simulink model "IEEE_BUS_68_Baseline"  (R2025a)
settings: Solver=ode23tb  StartTime=0.0  StopTime=150  FixedStep=Ts  MaxStep=0.0001  RelTol=1e-3
PreLoadFcn:
  | PSSMODEL=1;
  | LPSS=0;
  | WAPSS=0;
  | WAPSS2=0;
  | Ts=50e-5;
InitFcn:
  | PSSMODEL=1;
  | LPSS=0;
  | WAPSS=0;
  | WAPSS2=0;
  | Ts=50e-5;
  | 
  | % Required data to 68 Bus benchmark
  | % clear
  | % clc
  | % Definition for the columns
  | % system base =100 MVA
  | 
  | %% Line data Format (line)
  | % All values are given on the same system base MVA
  | % 1: From bus
  | % 2: To bus
  | % 3: Resistance (pu)
  | % 4: Reactance  (pu)
  | % 5: Charge     (pu)
  | % 6: Transformer Tap Amplitute
  | % 7: base MVA
  | % 8: Nomonal Voltage (KV)
  | 
  | %1   2    3        4       5       6        7      8
  | line=[...
  | 1	54	0	     0.0181	  0	      1.025     100    13.8
  | 2	58	0	     0.025	  0	      1.070     100    13.8
  | 3	62	0	     0.02	  0	      1.070     100    13.8
  | 4	19	0.0007	 0.0142	  0	      1.070     100    13.8
  | 5	20	0.0009	 0.018	  0	      1.009     100    13.8
  | 6	22	0	     0.0143	  0	      1.025     100    13.8
  | 7	23	0.0005	 0.0272	  0	      0         100    13.8
  | 8	25	0.0006	 0.0232	  0	      1.025     100    13.8
  | 9	29	0.0008	 0.0156   0	      1.025     100    13.8
  | 10	31	0	     0.026	  0	      1.04      100    13.8
  | 11	32	0	     0.013	  0	      1.04      100    13.8
  | 12	36	0	     0.0075	  0	      1.04      100    13.8
  | 13	17	0	     0.0033	  0	      1.04      100    13.8
  | 14	41	0	     0.0015	  0	      1         100    13.8
  | 15	42	0	     0.0015	  0	      1         100    13.8
  | 16	18	0	     0.003	  0	      1         100    13.8
  | 17	36	0.0005	 0.0045	  0.32	  0         100    138
  | 17	43	0.0005	 0.0276	  0	      0         100    138
  | 18	42	0.004	 0.06	  2.25    0         100    138
  | 18	49	0.0076	 0.1141	  1.16    0	        100    138
  | 18	50	0.0012	 0.0288	  2.06	  0         100    138
  | 20	19	0.0007	 0.0138	  0       1.06	    100    138
  | 19	68	0.0016	 0.0195	  0.304	  0         100    138
  | 21	22	0.0008	 0.014	  0.2565  0	        100    138
  | 21	68	0.0008	 0.0135	  0.2548  0	        100    138
  | 22	23	0.0006	 0.0096	  0.1846  0	        100    138
  | 23	24	0.0022	 0.035	  0.361	  0         100    138
  | 24	68	0.0003	 0.0059	  0.068	  0         100    138
  | 25	26	0.0032	 0.0323	  0.531	  0         100    138
  | 25	54	0.007	 0.0086	  0.146	  0         100    138
  | 26	27	0.0014	 0.0147	  0.2396  0	        100    138
  | 26	28	0.0043	 0.0474	  0.7802  0	        100    138
  | 26	29	0.0057	 0.0625	  1.029	  0         100    138
  | 27	37	0.0013	 0.0173	  0.3216  0	        100    138
  | 27	53	0.032	 0.32	  0.41	  0         100    138
  | ... (+206 lines)
undefined symbols (not defined in the file or in its folder): D1, Delta
libraries: spsRMSLib x73, spsThreePhaseVIMeasurementLib x69, spsLoadFlowBusLib x69, spsThreePhasePISectionLineLib x64, spsThreePhaseParallelRLCLoadLib x35, spsGenericPowerSystemStabilizerLib x32, spsThreePhaseSeriesRLCLoadLib x21, spsThreePhaseTransformerTwoWindingsLib x21, spsSynchronousMachinepuStandardLib x19, spsExcitationSystemLib x16, spsMultiBandPowerSystemStabilizerLib x16, spsSteamTurbineandGovernorLib x16
(part 7 of 7)

== system IEEE_BUS_68_Baseline/area-5/G15/M15: Turbine & Regulators  ==
  note: M15
  m15 : Inport
  Pref15 : Inport  Port=2
  Vref15 : Inport  Port=3
  PSS15 : Inport  Port=4
  Bus Selector : BusSelector  OutputSignals="Mechanical.Rotor speed  wm  (pu),Mechanical.Rotor angle deviation  d_theta (rad),Mechanical.Electrical power  Pe (pu),Mechanical.Rotor speed deviation  dw (pu),Mechanical.Rotor mechanical angle  theta (deg),dq0 components.Stator voltage  vd (pu),dq0 components.Stator voltage  vq (pu),Output reactive power  Qeo (pu)"
  "Delta Pa PSS 15 " : spsGenericPowerSystemStabilizerLib/Generic Power System Stabilizer  Tsensor=15e-3  K=2.5*1.25  Twashout=1  Tleadlag1=[60e-3 1]  Tleadlag2=[0 0]  VSlimits=[-0.15 0.15]  Vinit=0  Plot_On=off  MagdB_On=on  FreqRange=logspace(-2,2,500)
      settings: LibrarySourceBlock=|
      | sps_lib/Electrical Machines/Synchronous Machine Control/Generic
      | Power System Stabilizer
  Delta w PSS (Kundur) 15 : spsGenericPowerSystemStabilizerLib/Generic Power System Stabilizer  Tsensor=15e-3  K=30  Twashout=10  Tleadlag1=[50e-3 20e-3]  Tleadlag2=[3 5.4]  VSlimits=[-0.15 0.15]  Vinit=0  Plot_On=off  MagdB_On=on  FreqRange=logspace(-2,2,500)
      settings: LibrarySourceBlock=|
      | sps_lib/Electrical Machines/Synchronous Machine Control/Generic
      | Power System Stabilizer
  EXCITATION15 : spsExcitationSystemLib/Excitation System  tr=AVR_Data(16,1)  reg=[ AVR_Data(16,2:3) ]  exc=[ 1, 0 ]  tgr=[ AVR_Data(16,4:5)]  damp=[ 0, 0 ]  sat=[ 0, 0 ]  lim="[ AVR_Data(16,7:8)  0 ]"  v0=[1 1.0005]
      settings: LibrarySourceBlock=sps_lib/Electrical Machines/Synchronous Machine Control/Excitation System
  MB-PSS15 : spsMultiBandPowerSystemStabilizerLib/Multi-Band Power System Stabilizer  OperationMode=Simplified settings  Kg=MB(1)  GL=[MB(2) MB(3)]  GI=[MB(4) MB(5)]  GH=[MB(6) MB(7)]  GLd=[66 66 9.4]  TcLF=[1.667 2 0 0 0 0 2 2.4 0 0 0 0 1 1]  GId=[66 66 47.6]  TcIF=[1 1 0.25 0.3 0 0 1 1 0.3 0.36 0 0 0 0]  GHd=[66 66 233]  TcHF="[0.01 0.012 0 0 0 0  0.012 0.0144 0 0 0 0 1 1]"  LIM=[.075 .15 .15 .15]  Plot_On=off  MagdB_On=off  FreqRange=logspace(-2,2,500)
      settings: LibrarySourceBlock=|
      | sps_lib/Electrical Machines/Synchronous Machine Control/Multi-Band
      | Power System Stabilizer
  Multiport Switch1 : MultiPortSwitch  Inputs=4  SaturateOnIntegerOverflow=off
  PSS model3 : Constant  Value=0
  PSS model4 : Constant
  Real-Imag to Complex1 : RealImagToComplex
  STG15 : spsSteamTurbineandGovernorLib/Steam Turbine and Governor  gentype=Tandem-compound (single mass)  reg1="[ 1  0.05    0 ]"  reg2="[ 0.001  0.15 ]"  reg3="[ -0.1  0.1  0  4.496 ]"  N=Ns  turb1="[ 0  10   3.3   0.5   ]"  turb2="[   0   0.36    0.36   0.28   ]"  HA="[ 0.046  1.430  1.465   0.192 ]"  KA="[ 90.44  53.88  64.59   62.94  ]"  DA="[ 0.0115  0.3575  0.3663   0.0137  ]"  ini1=0.33333  ini2=[0.779316,-31.4247]
      settings: LibrarySourceBlock=|
      | sps_lib/Electrical Machines/Synchronous Machine Control/Steam Turbine
      | and Governor
  Sum2 : Sum  InputSameDT=on  SaturateOnIntegerOverflow=on  OutDataTypeStr=Inherit: Same as first input
  Sum3 : Sum  Inputs=-+  InputSameDT=on  SaturateOnIntegerOverflow=on  OutDataTypeStr=Inherit: Same as first input
  Terminator3 : Terminator
  Terminator4 : Terminator
  Terminator5 : Terminator
  wref15 : Constant
  Pm15 : Outport  InitialOutput=0
  Vf15 : Outport  Port=2  InitialOutput=0
  tag scope: EFD15=global, Pa15=global, Pe15=global, Q15=global, Vt15=global, d_theta15=global, pss15=global, theta15=global, w15=global
  wires:
  Bus Selector/7 -> EXCITATION15/3, Real-Imag to Complex1/2  "<Stator voltage  vq (pu)>"
  wref15/1 -> STG15/1
  Pref15/1 -> STG15/2
  m15/1 -> Bus Selector/1
  Vref15/1 -> EXCITATION15/1
  EXCITATION15/1 -> Vf15/1, [EFD15]
  Real-Imag to Complex1/1 -> [Vt15]
  Bus Selector/5 -> [theta15]  "<Rotor mechanical angle  theta (deg)>"
  Bus Selector/6 -> EXCITATION15/2, Real-Imag to Complex1/1  "<Stator voltage  vd (pu)>"
  STG15/3 -> Terminator3/1
  STG15/4 -> Sum3/2, Pm15/1
  STG15/2 -> Terminator4/1
  STG15/1 -> Terminator5/1
  Bus Selector/1 -> [w15], STG15/3  "<Rotor speed  wm  (pu)>"
  Bus Selector/2 -> STG15/4, [d_theta15]  "<Rotor angle deviation  d_theta (rad)>"
  Bus Selector/3 -> Sum3/1, [Pe15]  "<Electrical power  Pe (pu)>"
  Bus Selector/4 -> Delta w PSS (Kundur) 15/1, MB-PSS15/1  "<Rotor speed deviation  dw (pu)>"
  Bus Selector/8 -> [Q15]  "<Output reactive power  Qeo (pu)>"
  Sum3/1 -> [Pa15], "Delta Pa PSS 15 "/1  "Pm-Pe"
  Sum2/1 -> Multiport Switch1/1
  PSS model4/1 -> Sum2/2
  "Delta Pa PSS 15 "/1 -> Multiport Switch1/5
  Delta w PSS (Kundur) 15/1 -> Multiport Switch1/4
  MB-PSS15/1 -> Multiport Switch1/3
  PSS model3/1 -> Multiport Switch1/2
  Multiport Switch1/1 -> [pss15], EXCITATION15/4
  PSS15/1 -> Sum2/1

== system IEEE_BUS_68_Baseline/area-5/G16/M16: Turbine & Regulators  ==
  note: M16
  m16 : Inport
  Pref16 : Inport  Port=2
  Vref16 : Inport  Port=3
  PSS16 : Inport  Port=4
  Bus Selector : BusSelector  OutputSignals="Mechanical.Rotor speed  wm  (pu),Mechanical.Rotor angle deviation  d_theta (rad),Mechanical.Electrical power  Pe (pu),Mechanical.Rotor speed deviation  dw (pu),Mechanical.Rotor mechanical angle  theta (deg),dq0 components.Stator voltage  vd (pu),dq0 components.Stator voltage  vq (pu),Output reactive power  Qeo (pu)"
  "Delta Pa PSS 16 " : spsGenericPowerSystemStabilizerLib/Generic Power System Stabilizer  Tsensor=15e-3  K=2.5*1.25  Twashout=1  Tleadlag1=[60e-3 1]  Tleadlag2=[0 0]  VSlimits=[-0.15 0.15]  Vinit=0  Plot_On=off  MagdB_On=on  FreqRange=logspace(-2,2,500)
      settings: LibrarySourceBlock=|
      | sps_lib/Electrical Machines/Synchronous Machine Control/Generic
      | Power System Stabilizer
  Delta w PSS (Kundur) 16 : spsGenericPowerSystemStabilizerLib/Generic Power System Stabilizer  Tsensor=15e-3  K=30  Twashout=10  Tleadlag1=[50e-3 20e-3]  Tleadlag2=[3 5.4]  VSlimits=[-0.15 0.15]  Vinit=0  Plot_On=off  MagdB_On=on  FreqRange=logspace(-2,2,500)
      settings: LibrarySourceBlock=|
      | sps_lib/Electrical Machines/Synchronous Machine Control/Generic
      | Power System Stabilizer
  EXCITATION16 : spsExcitationSystemLib/Excitation System  tr=AVR_Data(13,1)  reg=[ AVR_Data(13,2:3) ]  exc=[ 1, 0 ]  tgr=[ AVR_Data(13,4:5)]  damp=[ 0, 0 ]  sat=[ 0, 0 ]  lim="[ AVR_Data(13,7:8)  0 ]"  v0=[1 1.0013]
      settings: LibrarySourceBlock=sps_lib/Electrical Machines/Synchronous Machine Control/Excitation System
  MB-PSS16 : spsMultiBandPowerSystemStabilizerLib/Multi-Band Power System Stabilizer  OperationMode=Simplified settings  Kg=MB(1)  GL=[MB(2) MB(3)]  GI=[MB(4) MB(5)]  GH=[MB(6) MB(7)]  GLd=[66 66 9.4]  TcLF=[1.667 2 0 0 0 0 2 2.4 0 0 0 0 1 1]  GId=[66 66 47.6]  TcIF=[1 1 0.25 0.3 0 0 1 1 0.3 0.36 0 0 0 0]  GHd=[66 66 233]  TcHF="[0.01 0.012 0 0 0 0  0.012 0.0144 0 0 0 0 1 1]"  LIM=[.075 .15 .15 .15]  Plot_On=off  MagdB_On=off  FreqRange=logspace(-2,2,500)
      settings: LibrarySourceBlock=|
      | sps_lib/Electrical Machines/Synchronous Machine Control/Multi-Band
      | Power System Stabilizer
  Multiport Switch1 : MultiPortSwitch  Inputs=4  SaturateOnIntegerOverflow=off
  PSS model3 : Constant  Value=0
  PSS model4 : Constant
  Real-Imag to Complex1 : RealImagToComplex
  STG13 : spsSteamTurbineandGovernorLib/Steam Turbine and Governor  gentype=Tandem-compound (single mass)  reg1="[ 1  0.05    0 ]"  reg2="[ 0.001  0.15 ]"  reg3="[ -0.1  0.1  0  4.496 ]"  N=Ns  turb1="[ 0  10   3.3   0.5   ]"  turb2="[   0   0.36    0.36   0.28   ]"  HA="[ 0.046  1.430  1.465   0.192 ]"  KA="[ 90.44  53.88  64.59   62.94  ]"  DA="[ 0.0115  0.3575  0.3663   0.0137  ]"  ini1=0.58333  ini2=[0.779316,-31.4247]
      settings: LibrarySourceBlock=|
      | sps_lib/Electrical Machines/Synchronous Machine Control/Steam Turbine
      | and Governor
  Sum2 : Sum  InputSameDT=on  SaturateOnIntegerOverflow=on  OutDataTypeStr=Inherit: Same as first input
  Sum3 : Sum  Inputs=-+  InputSameDT=on  SaturateOnIntegerOverflow=on  OutDataTypeStr=Inherit: Same as first input
  Terminator3 : Terminator
  Terminator4 : Terminator
  Terminator5 : Terminator
  wref16 : Constant
  Pm16 : Outport  InitialOutput=0
  Vf16 : Outport  Port=2  InitialOutput=0
  tag scope: EFD16=global, Pa16=global, Pe16=global, Q16=global, Vt16=global, d_theta16=global, pss16=global, theta16=global, w16=global
  wires:
  PSS16/1 -> Sum2/1
  Multiport Switch1/1 -> EXCITATION16/4, [pss16]
  PSS model3/1 -> Multiport Switch1/2
  MB-PSS16/1 -> Multiport Switch1/3
  Delta w PSS (Kundur) 16/1 -> Multiport Switch1/4
  "Delta Pa PSS 16 "/1 -> Multiport Switch1/5
  PSS model4/1 -> Sum2/2
  Sum2/1 -> Multiport Switch1/1
  Sum3/1 -> "Delta Pa PSS 16 "/1, [Pa16]  "Pm-Pe"
  Bus Selector/8 -> [Q16]  "<Output reactive power  Qeo (pu)>"
  Bus Selector/4 -> MB-PSS16/1, Delta w PSS (Kundur) 16/1  "<Rotor speed deviation  dw (pu)>"
  Bus Selector/3 -> [Pe16], Sum3/1  "<Electrical power  Pe (pu)>"
  Bus Selector/2 -> [d_theta16], STG13/4  "<Rotor angle deviation  d_theta (rad)>"
  Bus Selector/1 -> STG13/3, [w16]  "<Rotor speed  wm  (pu)>"
  STG13/1 -> Terminator5/1
  STG13/2 -> Terminator4/1
  STG13/4 -> Pm16/1, Sum3/2
  STG13/3 -> Terminator3/1
  Bus Selector/6 -> Real-Imag to Complex1/1, EXCITATION16/2  "<Stator voltage  vd (pu)>"
  Bus Selector/5 -> [theta16]  "<Rotor mechanical angle  theta (deg)>"
  Real-Imag to Complex1/1 -> [Vt16]
  EXCITATION16/1 -> [EFD16], Vf16/1
  Vref16/1 -> EXCITATION16/1
  m16/1 -> Bus Selector/1
  Pref16/1 -> STG13/2
  wref16/1 -> STG13/1
  Bus Selector/7 -> Real-Imag to Complex1/2, EXCITATION16/3  "<Stator voltage  vq (pu)>"
